simulink subsystem "piero_modelZ"  (R2022b)
settings: Solver=VariableStepAuto  StartTime=0.0  StopTime=10.0  RelTol=1e-3
settings Model: Creator=miriamfreiriasanjuan  LastModifiedBy=miriamfreiriasanjuan

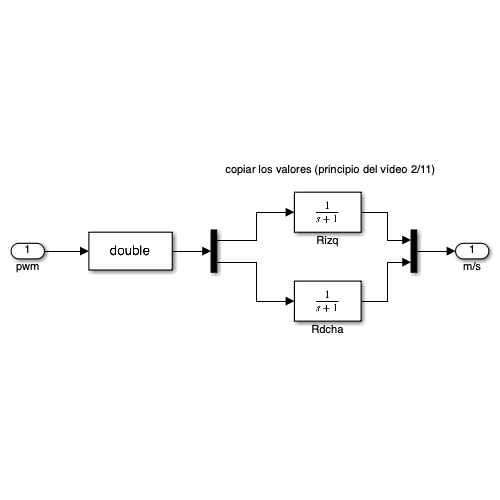
[thumbnail: Simulink's stored preview of the top-level diagram]
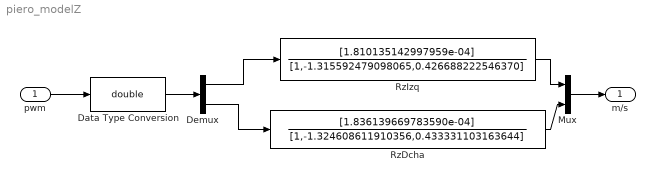
== system piero_modelZ ==
  pwm : Inport
  Data Type Conversion : DataTypeConversion  OutDataTypeStr=double  SaturateOnIntegerOverflow=off  RndMeth=Floor
  Demux : Demux  Outputs=2
  Mux : Mux  Inputs=2
  RzDcha : DiscreteFilter  Numerator=[1.836139669783590e-04]  Denominator=[1,-1.324608611910356,0.433331103163644]
  RzIzq : DiscreteFilter  Numerator=[1.810135142997959e-04]  Denominator=[1,-1.315592479098065,0.426688222546370]
  m/s : Outport
  wires:
  pwm/1 -> Data Type Conversion/1
  Mux/1 -> m/s/1
  Demux/1 -> RzIzq/1
  Demux/2 -> RzDcha/1
  RzIzq/1 -> Mux/1
  RzDcha/1 -> Mux/2
  Data Type Conversion/1 -> Demux/1
